simulink model "afe_inv_ttype_psm"  (R2026a)
settings: Solver=ode23tb  StopTime=simlength  FixedStep=tc  MaxStep=glb_time.tc
values from neighbouring files (symbols this model uses):
  afe_ctrl = ctrl_afe_setup(glb_time.ts_afe, grid_emu.omega_grid_nom)    [init_model.m]
  afe_pwm_phase_shift_mod1 = 0    [init_model.m]
  DThs_init = 0    [init_model.m]
  filters = setup_global_filters(glb_time.ts_afe, glb_time.ts_inv, glb_time.ts_dab, glb_time.tc)    [init_model.m]
  frt_data = frt_settings(test_index, test_subindex, asymmetric_error_type,      enable_frt_1, enable_frt_2, start_time_LVRT, deepPOSxi, deepPOSeta, deepNEGxi, deepNEGeta)    [init_model.m]
  glb_time = timing_setup(fpwm_afe, trgo_afe, fpwm_inv, trgo_inv, fpwm_single_phase_inv, trgo_single_phase_inv, fpwm_dab, trgo_dab,      fpwm_psfbc, trgo_psfbc, fpwm_isop_rail, trgo_isop_rail, fpwm_cllc, trgo_cllc, t_measure, tc_factor, tc_decimation, delay_pwm, dead_time_afe,      dead_time_inv, dead_time_single_phase_inv, dead_time_dab, dead_time_psfbc, dead_time_isop_rail, dead_time_cllc)    [init_model.m]
  grid_emu = grid_three_phase_emulator('Dyn11', delta_star, grid_nominal_power, application_voltage, us1, us2, fgrid,                  eq_grid_inductance, eq_grid_resistance, eta, ucc, i1m, p_iron, n1, n2, core_area, core_length, mur,                  up_xi_pu_ref, up_eta_pu_ref, un_xi_pu_ref, un_eta_pu_ref)    [init_model.m]
  i_react_pos_ref_2 = -ixi_ref_mod1*tan(acos(0.95))    [init_model.m]
  i_react_pos_ref_3 = ixi_ref_mod1*tan(acos(0.95))    [init_model.m]
  ixi_ref_mod1 = -0.85    [init_model.m]
  ki_align = 18    [init_model.m]
  kp_align = 0.25    [init_model.m]
  lim_down_align = -0.05    [init_model.m]
  lim_up_align = 0.05    [init_model.m]
  mavarage_filter_frequency_base_order = 2    [init_model.m]
  omega_m_sim = psm.omega_m_bez    [init_model.m]
  psm = psm_calculus()    [init_model.m]
  psm_ctrl = ctrl_pmsm_setup(glb_time.ts_inv, psm.omega_bez, u_psm_scale, psm.Jm_norm)    [init_model.m]
  simlength = 1.75    [init_model.m]
  Tambient = 40    [init_model.m]
  time_aux_power_supply_fault = 1e3    (= 1000)    [init_model.m]
  time_gain_afe_module_1 = 1.0002    [init_model.m]
  time_gain_inv_module_2 = 1.001    [init_model.m]
  time_i_react_pos_ref_1 = start_time_LVRT + error_length + 0.335    [init_model.m]
  time_i_react_pos_ref_2 = time_i_react_pos_ref_1 + 0.5    (= 0.5)    [init_model.m]
  time_start_motor_control = 0.25    [init_model.m]
  torque_overload_factor = 1    [init_model.m]
  u_cm_comp_mod1 = 0    [init_model.m]
  u_psm_scale_ekf = sqrt(3)/2 * 2/3 * hwdata.inv.udc_nom/psm.ubez    [init_model.m]
undefined symbols (not defined in the file or in its folder): hwdata, magnitude, omega_m_bez, rpm_base, torque_base
libraries: fl_lib x74, nesl_utility x43, moving_average_filter x10, moving_average_filter_cc x8, discrete_time_low_pass_filter x4, sl_discontinuities x3, single_phase_transformer_lib x3, linear_double_integrator_observer_ccaller x2, threephase_inductor_lib x2, dclink_for_three_levels x2, three_phase_three_level_ttype_inverter_ideal_switch_based_model x2, cstblocks_lti x2
(part 6 of 9)

== system afe_inv_ttype_psm/afe_abc_inv_psm_mod1/AFE_control/afe_control/grid_voltage_phase_lock_loops/dq_pll_ccaller/first_harmonic_tracker_phase_u ==
  u : Inport
  Bus Selector : BusSelector  OutputSignals=output_pu_hat
  C Caller : CCaller  FunctionName=first_harmonic_tracker_process_simulink  PortSpecificationStruct="%)30     .    B \\   8    (     @         %    \"     D    !     0         %  0 \"0    $    _    07)G3F%M90  4&]R=$YA;64 4V-O<&4     26YD97@     5'EP90      4VEZ90      27-';&]B86P   X    P    !@    @    $          4    (     0    ,    !         !   P!O=70 #@   #     &    \"     0         !0    @    !     P    $         $  # &]U=  .    .     8    (    !          %    \"     $    &     0         0  ...(+4988 chars)"
  Constant : Constant  Value=glb_time.ts_afe
  Constant1 : Constant  Value=0
  Constant4 : Constant  Value=afe_ctrl.fht_grid.omega_fht
  Constant5 : Constant  Value=afe_ctrl.fht_grid.delta_fht
  Constant6 : Constant  Value=afe_ctrl.fht_grid.Ld_fht(1)
  Constant7 : Constant  Value=afe_ctrl.fht_grid.Ld_fht(2)
  Data Type Conversion{1..2,6..9} (6 alike) : DataTypeConversion  OutDataTypeStr=single  SaturateOnIntegerOverflow=off  RndMeth=Floor
  Data Type Conversion3 : DataTypeConversion  OutDataTypeStr=uint8  SaturateOnIntegerOverflow=off  RndMeth=Floor
  Data Type Conversion4 : DataTypeConversion  OutDataTypeStr=double  SaturateOnIntegerOverflow=off  RndMeth=Floor
  Data Type Conversion5 : DataTypeConversion  OutDataTypeStr=uint8  SaturateOnIntegerOverflow=off  RndMeth=Floor
  Step : Step  Time=0.0125  InitialValue=1  FinalValue=0
  u_hat : Outport
  wires:
  Data Type Conversion4/1 -> u_hat/1
  Data Type Conversion3/1 -> C Caller/1
  Data Type Conversion1/1 -> C Caller/3
  Data Type Conversion2/1 -> C Caller/2
  C Caller/1 -> Bus Selector/1
  Bus Selector/1 -> Data Type Conversion4/1  "<output_pu_hat>"
  Step/1 -> Data Type Conversion3/1
  u/1 -> Data Type Conversion2/1
  Constant/1 -> Data Type Conversion1/1
  Constant1/1 -> Data Type Conversion5/1
  Constant4/1 -> Data Type Conversion6/1
  Constant6/1 -> Data Type Conversion8/1
  Constant7/1 -> Data Type Conversion9/1
  Constant5/1 -> Data Type Conversion7/1
  Data Type Conversion5/1 -> C Caller/8
  Data Type Conversion6/1 -> C Caller/4
  Data Type Conversion7/1 -> C Caller/5
  Data Type Conversion8/1 -> C Caller/6
  Data Type Conversion9/1 -> C Caller/7

== system afe_inv_ttype_psm/afe_abc_inv_psm_mod1/AFE_control/afe_control/grid_voltage_phase_lock_loops/dq_pll_ccaller/first_harmonic_tracker_phase_v ==
  u : Inport
  Bus Selector : BusSelector  OutputSignals=output_pu_hat
  C Caller : CCaller  FunctionName=first_harmonic_tracker_process_simulink  PortSpecificationStruct="%)30     .    B \\   8    (     @         %    \"     D    !     0         %  0 \"0    $    _    07)G3F%M90  4&]R=$YA;64 4V-O<&4     26YD97@     5'EP90      4VEZ90      27-';&]B86P   X    P    !@    @    $          4    (     0    ,    !         !   P!O=70 #@   #     &    \"     0         !0    @    !     P    $         $  # &]U=  .    .     8    (    !          %    \"     $    &     0         0  ...(+4988 chars)"
  Constant : Constant  Value=glb_time.ts_afe
  Constant1 : Constant  Value=2
  Constant4 : Constant  Value=afe_ctrl.fht_grid.omega_fht
  Constant5 : Constant  Value=afe_ctrl.fht_grid.delta_fht
  Constant6 : Constant  Value=afe_ctrl.fht_grid.Ld_fht(1)
  Constant7 : Constant  Value=afe_ctrl.fht_grid.Ld_fht(2)
  Data Type Conversion{1..2,6..9} (6 alike) : DataTypeConversion  OutDataTypeStr=single  SaturateOnIntegerOverflow=off  RndMeth=Floor
  Data Type Conversion3 : DataTypeConversion  OutDataTypeStr=uint8  SaturateOnIntegerOverflow=off  RndMeth=Floor
  Data Type Conversion4 : DataTypeConversion  OutDataTypeStr=double  SaturateOnIntegerOverflow=off  RndMeth=Floor
  Data Type Conversion5 : DataTypeConversion  OutDataTypeStr=uint8  SaturateOnIntegerOverflow=off  RndMeth=Floor
  Step : Step  Time=0.0125  InitialValue=1  FinalValue=0
  u_hat : Outport
  wires:
  Data Type Conversion9/1 -> C Caller/7
  Data Type Conversion8/1 -> C Caller/6
  Data Type Conversion7/1 -> C Caller/5
  Data Type Conversion6/1 -> C Caller/4
  Data Type Conversion5/1 -> C Caller/8
  Constant5/1 -> Data Type Conversion7/1
  Constant7/1 -> Data Type Conversion9/1
  Constant6/1 -> Data Type Conversion8/1
  Constant4/1 -> Data Type Conversion6/1
  Constant1/1 -> Data Type Conversion5/1
  Constant/1 -> Data Type Conversion1/1
  u/1 -> Data Type Conversion2/1
  Step/1 -> Data Type Conversion3/1
  Bus Selector/1 -> Data Type Conversion4/1  "<output_pu_hat>"
  C Caller/1 -> Bus Selector/1
  Data Type Conversion2/1 -> C Caller/2
  Data Type Conversion1/1 -> C Caller/3
  Data Type Conversion3/1 -> C Caller/1
  Data Type Conversion4/1 -> u_hat/1

== system afe_inv_ttype_psm/afe_abc_inv_psm_mod1/AFE_control/afe_control/grid_voltage_phase_lock_loops/dq_pll_ccaller/first_harmonic_tracker_phase_w ==
  u : Inport
  Bus Selector : BusSelector  OutputSignals=output_pu_hat
  C Caller : CCaller  FunctionName=first_harmonic_tracker_process_simulink  PortSpecificationStruct="%)30     .    B \\   8    (     @         %    \"     D    !     0         %  0 \"0    $    _    07)G3F%M90  4&]R=$YA;64 4V-O<&4     26YD97@     5'EP90      4VEZ90      27-';&]B86P   X    P    !@    @    $          4    (     0    ,    !         !   P!O=70 #@   #     &    \"     0         !0    @    !     P    $         $  # &]U=  .    .     8    (    !          %    \"     $    &     0         0  ...(+4988 chars)"
  Constant : Constant  Value=glb_time.ts_afe
  Constant1 : Constant  Value=4
  Constant4 : Constant  Value=afe_ctrl.fht_grid.omega_fht
  Constant5 : Constant  Value=afe_ctrl.fht_grid.delta_fht
  Constant6 : Constant  Value=afe_ctrl.fht_grid.Ld_fht(1)
  Constant7 : Constant  Value=afe_ctrl.fht_grid.Ld_fht(2)
  Data Type Conversion{1..2,6..9} (6 alike) : DataTypeConversion  OutDataTypeStr=single  SaturateOnIntegerOverflow=off  RndMeth=Floor
  Data Type Conversion3 : DataTypeConversion  OutDataTypeStr=uint8  SaturateOnIntegerOverflow=off  RndMeth=Floor
  Data Type Conversion4 : DataTypeConversion  OutDataTypeStr=double  SaturateOnIntegerOverflow=off  RndMeth=Floor
  Data Type Conversion5 : DataTypeConversion  OutDataTypeStr=uint8  SaturateOnIntegerOverflow=off  RndMeth=Floor
  Step : Step  Time=0.0125  InitialValue=1  FinalValue=0
  u_hat : Outport
  wires:
  Data Type Conversion4/1 -> u_hat/1
  Data Type Conversion3/1 -> C Caller/1
  Data Type Conversion1/1 -> C Caller/3
  Data Type Conversion2/1 -> C Caller/2
  C Caller/1 -> Bus Selector/1
  Bus Selector/1 -> Data Type Conversion4/1  "<output_pu_hat>"
  Step/1 -> Data Type Conversion3/1
  u/1 -> Data Type Conversion2/1
  Constant/1 -> Data Type Conversion1/1
  Constant1/1 -> Data Type Conversion5/1
  Constant4/1 -> Data Type Conversion6/1
  Constant6/1 -> Data Type Conversion8/1
  Constant7/1 -> Data Type Conversion9/1
  Constant5/1 -> Data Type Conversion7/1
  Data Type Conversion5/1 -> C Caller/8
  Data Type Conversion6/1 -> C Caller/4
  Data Type Conversion7/1 -> C Caller/5
  Data Type Conversion8/1 -> C Caller/6
  Data Type Conversion9/1 -> C Caller/7

== system afe_inv_ttype_psm/afe_abc_inv_psm_mod1/AFE_control/afe_control/grid_voltage_sequences/voltage_sequence_avg/average_filter ==
  v_grid_pos_xi : Inport
  v_grid_pos_eta : Inport  Port=2
  v_grid_neg_xi : Inport  Port=3
  v_grid_neg_eta : Inport  Port=4
  Abs : Abs  SaturateOnIntegerOverflow=off
  Gain : Gain  Gain=grid_emu.omega_grid_nom*mavarage_filter_frequency_base_order
  Saturation : Saturate  UpperLimit=2  LowerLimit=0.1
  dmavg_flt{,1..3} (4 alike) : moving_average_filter/dmavg_flt  ts=glb_time.ts_afe  enable_time=dmavg_filter_enable_time
  v_grid_pos_xi_avg : Outport
  v_grid_pos_eta_avg : Outport  Port=2
  v_grid_neg_xi_avg : Outport  Port=3
  v_grid_neg_eta_avg : Outport  Port=4
  wires:
  v_grid_neg_eta/1 -> dmavg_flt3/1
  v_grid_neg_xi/1 -> dmavg_flt2/1
  v_grid_pos_eta/1 -> dmavg_flt1/1
  dmavg_flt3/1 -> v_grid_neg_eta_avg/1
  dmavg_flt2/1 -> v_grid_neg_xi_avg/1
  dmavg_flt1/1 -> v_grid_pos_eta_avg/1
  Gain/1 -> dmavg_flt/2, dmavg_flt1/2, dmavg_flt2/2, dmavg_flt3/2
  dmavg_flt/1 -> v_grid_pos_xi_avg/1
  v_grid_pos_xi/1 -> dmavg_flt/1
  Abs/1 -> Saturation/1
  [omega_grid_pll_pu] -> Abs/1
  Saturation/1 -> Gain/1

== system afe_inv_ttype_psm/afe_abc_inv_psm_mod1/AFE_control/afe_control/grid_voltage_sequences/voltage_sequence_avg/average_filter_ccaller ==
  v_grid_pos_xi : Inport
  v_grid_pos_eta : Inport  Port=2
  v_grid_neg_xi : Inport  Port=3
  v_grid_neg_eta : Inport  Port=4
  Abs : Abs  SaturateOnIntegerOverflow=off
  Gain : Gain  Gain=grid_emu.omega_grid_nom*mavarage_filter_frequency_base_order
  Saturation : Saturate  UpperLimit=2  LowerLimit=0.1
  dmavg_flt : moving_average_filter_cc/dmavg_flt  instance=0  ts=glb_time.ts_afe  enable_time=dmavg_filter_enable_time
  dmavg_flt1 : moving_average_filter_cc/dmavg_flt  instance=1  ts=glb_time.ts_afe  enable_time=dmavg_filter_enable_time
  dmavg_flt2 : moving_average_filter_cc/dmavg_flt  instance=2  ts=glb_time.ts_afe  enable_time=dmavg_filter_enable_time
  dmavg_flt3 : moving_average_filter_cc/dmavg_flt  instance=3  ts=glb_time.ts_afe  enable_time=dmavg_filter_enable_time
  v_grid_pos_xi_avg : Outport
  v_grid_pos_eta_avg : Outport  Port=2
  v_grid_neg_xi_avg : Outport  Port=3
  v_grid_neg_eta_avg : Outport  Port=4
  wires:
  v_grid_pos_xi/1 -> dmavg_flt/1
  dmavg_flt/1 -> v_grid_pos_xi_avg/1
  dmavg_flt1/1 -> v_grid_pos_eta_avg/1
  dmavg_flt2/1 -> v_grid_neg_xi_avg/1
  dmavg_flt3/1 -> v_grid_neg_eta_avg/1
  v_grid_pos_eta/1 -> dmavg_flt1/1
  v_grid_neg_xi/1 -> dmavg_flt2/1
  v_grid_neg_eta/1 -> dmavg_flt3/1
  Abs/1 -> Saturation/1
  Saturation/1 -> Gain/1
  [omega_grid_pll_pu] -> Abs/1
  Gain/1 -> dmavg_flt/2, dmavg_flt1/2, dmavg_flt3/2, dmavg_flt2/2

== system afe_inv_ttype_psm/afe_abc_inv_psm_mod1/AFE_control/afe_control/phase_compensation_1/alignment_eval_afe1/pi ==
  u_ref : Inport
  u : Inport  Port=2
  1/Ti : Gain  Gain=kp  SaturateOnIntegerOverflow=on  OutDataTypeStr=Inherit: Same as input  ParamDataTypeStr=Inherit: Same as input
  Saturation : Saturate  UpperLimit=lim_up  LowerLimit=lim_down
  Sum1 : Sum  Inputs=+++  SaturateOnIntegerOverflow=on
  Sum2 : Sum  Inputs=-+  SaturateOnIntegerOverflow=on
  Sum3 : Sum  Inputs=-+  SaturateOnIntegerOverflow=on
  Unit Delay4 : UnitDelay  SampleTime=-1
  kp : Gain  Gain=ki  SaturateOnIntegerOverflow=on  OutDataTypeStr=Inherit: Same as input  ParamDataTypeStr=Inherit: Same as input
  y : Outport
  wires:
  1/Ti/1 -> Sum1/1, Sum3/1
  kp/1 -> Sum1/2
  Sum3/1 -> Unit Delay4/1
  Unit Delay4/1 -> Sum1/3
  u_ref/1 -> Sum2/2
  u/1 -> Sum2/1
  Sum2/1 -> kp/1, 1/Ti/1
  Sum1/1 -> Saturation/1
  Saturation/1 -> Sum3/2, y/1

== system afe_inv_ttype_psm/afe_abc_inv_psm_mod1/inv_psm_mod1/inverter/deadtime_generator_for_ttype/dead_time_generator_cmos_simulink_phu/dead_time_leg_generator_1 ==
  cmd_in_QA : Inport
  cmd_in_QB : Inport  Port=2
  MATLAB Function : MATLAB Function  TreatAsAtomicUnit=on
  MATLAB Function1 : MATLAB Function  TreatAsAtomicUnit=on
  MATLAB Function2 : MATLAB Function  TreatAsAtomicUnit=on
  MATLAB Function3 : MATLAB Function  TreatAsAtomicUnit=on
  MATLAB Function4 : MATLAB Function  TreatAsAtomicUnit=on
  MATLAB Function5 : MATLAB Function  TreatAsAtomicUnit=on
  MATLAB Function6 : MATLAB Function  TreatAsAtomicUnit=on
  MATLAB Function7 : MATLAB Function  TreatAsAtomicUnit=on
  MATLAB Function8 : MATLAB Function  TreatAsAtomicUnit=on
  MATLAB Function9 : MATLAB Function  TreatAsAtomicUnit=on
  Transfer Fcn : TransferFcn  Denominator=[sqrt(2)*deadtime 1]
  Transfer Fcn1 : TransferFcn  Denominator=[sqrt(2)*deadtime 1]
  cmd_out_QA : Outport
  cmd_out_QB : Outport  Port=2
  wires:
  MATLAB Function8/1(y) -> MATLAB Function5/2(u2)
  MATLAB Function7/1(y) -> Transfer Fcn1/1, MATLAB Function9/2(u2)
  MATLAB Function3/1(y) -> MATLAB Function1/2(u2)
  MATLAB Function2/1(y) -> Transfer Fcn/1, MATLAB Function4/1(u1)
  MATLAB Function/1(y) -> MATLAB Function1/1(u1), MATLAB Function2/1(u)
  MATLAB Function9/1(y) -> cmd_out_QB/1
  MATLAB Function4/1(y) -> cmd_out_QA/1
  MATLAB Function6/1(y) -> MATLAB Function5/1(u1), MATLAB Function7/1(u)
  cmd_in_QA/1 -> MATLAB Function/1(u)
  MATLAB Function5/1(y) -> MATLAB Function4/2(u2)
  MATLAB Function1/1(y) -> MATLAB Function9/1(u1)
  cmd_in_QB/1 -> MATLAB Function6/1(u)
  Transfer Fcn1/1 -> MATLAB Function8/1(u)
  Transfer Fcn/1 -> MATLAB Function3/1(u)

== system afe_inv_ttype_psm/afe_abc_inv_psm_mod1/inv_psm_mod1/inverter/deadtime_generator_for_ttype/dead_time_generator_cmos_simulink_phv/dead_time_leg_generator_1 ==
  cmd_in_QA : Inport
  cmd_in_QB : Inport  Port=2
  MATLAB Function : MATLAB Function  TreatAsAtomicUnit=on
  MATLAB Function1 : MATLAB Function  TreatAsAtomicUnit=on
  MATLAB Function2 : MATLAB Function  TreatAsAtomicUnit=on
  MATLAB Function3 : MATLAB Function  TreatAsAtomicUnit=on
  MATLAB Function4 : MATLAB Function  TreatAsAtomicUnit=on
  MATLAB Function5 : MATLAB Function  TreatAsAtomicUnit=on
  MATLAB Function6 : MATLAB Function  TreatAsAtomicUnit=on
  MATLAB Function7 : MATLAB Function  TreatAsAtomicUnit=on
  MATLAB Function8 : MATLAB Function  TreatAsAtomicUnit=on
  MATLAB Function9 : MATLAB Function  TreatAsAtomicUnit=on
  Transfer Fcn : TransferFcn  Denominator=[sqrt(2)*deadtime 1]
  Transfer Fcn1 : TransferFcn  Denominator=[sqrt(2)*deadtime 1]
  cmd_out_QA : Outport
  cmd_out_QB : Outport  Port=2
  wires:
  Transfer Fcn/1 -> MATLAB Function3/1(u)
  Transfer Fcn1/1 -> MATLAB Function8/1(u)
  cmd_in_QB/1 -> MATLAB Function6/1(u)
  MATLAB Function1/1(y) -> MATLAB Function9/1(u1)
  MATLAB Function5/1(y) -> MATLAB Function4/2(u2)
  cmd_in_QA/1 -> MATLAB Function/1(u)
  MATLAB Function6/1(y) -> MATLAB Function7/1(u), MATLAB Function5/1(u1)
  MATLAB Function4/1(y) -> cmd_out_QA/1
  MATLAB Function9/1(y) -> cmd_out_QB/1
  MATLAB Function/1(y) -> MATLAB Function2/1(u), MATLAB Function1/1(u1)
  MATLAB Function2/1(y) -> MATLAB Function4/1(u1), Transfer Fcn/1
  MATLAB Function3/1(y) -> MATLAB Function1/2(u2)
  MATLAB Function7/1(y) -> MATLAB Function9/2(u2), Transfer Fcn1/1
  MATLAB Function8/1(y) -> MATLAB Function5/2(u2)

== system afe_inv_ttype_psm/afe_abc_inv_psm_mod1/inv_psm_mod1/inverter/deadtime_generator_for_ttype/dead_time_generator_cmos_simulink_phw/dead_time_leg_generator_1 ==
  cmd_in_QA : Inport
  cmd_in_QB : Inport  Port=2
  MATLAB Function : MATLAB Function  TreatAsAtomicUnit=on
  MATLAB Function1 : MATLAB Function  TreatAsAtomicUnit=on
  MATLAB Function2 : MATLAB Function  TreatAsAtomicUnit=on
  MATLAB Function3 : MATLAB Function  TreatAsAtomicUnit=on
  MATLAB Function4 : MATLAB Function  TreatAsAtomicUnit=on
  MATLAB Function5 : MATLAB Function  TreatAsAtomicUnit=on
  MATLAB Function6 : MATLAB Function  TreatAsAtomicUnit=on
  MATLAB Function7 : MATLAB Function  TreatAsAtomicUnit=on
  MATLAB Function8 : MATLAB Function  TreatAsAtomicUnit=on
  MATLAB Function9 : MATLAB Function  TreatAsAtomicUnit=on
  Transfer Fcn : TransferFcn  Denominator=[sqrt(2)*deadtime 1]
  Transfer Fcn1 : TransferFcn  Denominator=[sqrt(2)*deadtime 1]
  cmd_out_QA : Outport
  cmd_out_QB : Outport  Port=2
  wires:
  MATLAB Function8/1(y) -> MATLAB Function5/2(u2)
  MATLAB Function7/1(y) -> Transfer Fcn1/1, MATLAB Function9/2(u2)
  MATLAB Function3/1(y) -> MATLAB Function1/2(u2)
  MATLAB Function2/1(y) -> Transfer Fcn/1, MATLAB Function4/1(u1)
  MATLAB Function/1(y) -> MATLAB Function1/1(u1), MATLAB Function2/1(u)
  MATLAB Function9/1(y) -> cmd_out_QB/1
  MATLAB Function4/1(y) -> cmd_out_QA/1
  MATLAB Function6/1(y) -> MATLAB Function5/1(u1), MATLAB Function7/1(u)
  cmd_in_QA/1 -> MATLAB Function/1(u)
  MATLAB Function5/1(y) -> MATLAB Function4/2(u2)
  MATLAB Function1/1(y) -> MATLAB Function9/1(u1)
  cmd_in_QB/1 -> MATLAB Function6/1(u)
  Transfer Fcn1/1 -> MATLAB Function8/1(u)
  Transfer Fcn/1 -> MATLAB Function3/1(u)

== system afe_inv_ttype_psm/afe_abc_inv_psm_mod1/inv_psm_mod1/inverter_ctrl/inverter_control/encoder-sensorless-switch/double_integrator_observer ==
  phase_psm : Inport
  Dead Zone : DeadZone  LowerValue=-0.01  UpperValue=0.01
  Gain : Gain  Gain=psm_ctrl.di_obs.komega
  Gain1 : Gain  Gain=psm_ctrl.di_obs.ktheta
  Gain2 : Gain  Gain=psm_ctrl.omega_base
  Gain3 : Gain  Gain=1/psm_ctrl.omega_base
  Gain4 : Gain  Gain=glb_time.ts_inv
  Gain5 : Gain  Gain=glb_time.ts_inv
  Gain6 : Gain  Gain=glb_time.ts_inv
  Sum : Sum  Inputs=-+|
  Sum1 : Sum  Inputs=|++
  Sum2 : Sum  Inputs=|++
  Sum8 : Sum  Inputs=++|
  Unit Delay1 : UnitDelay  InitialCondition=pi  SampleTime=-1
  Unit Delay2 : UnitDelay  SampleTime=-1
  bounder1 : MATLAB Function  TreatAsAtomicUnit=on
  bounder2 : MATLAB Function  TreatAsAtomicUnit=on
  omega_pu_psm_hat : Outport  VectorParamsAs1DForOutWhenUnconnected=off
  phase_psm_hat : Outport  Port=2  VectorParamsAs1DForOutWhenUnconnected=off
  wires:
  Gain1/1 -> Gain6/1
  phase_psm/1 -> Sum/2
  Sum8/1 -> Unit Delay1/1
  Unit Delay1/1 -> bounder2/1(u)
  Sum1/1 -> Unit Delay2/1
  Gain/1 -> Gain4/1
  Unit Delay2/1 -> omega_pu_psm_hat/1, Sum1/2, Gain5/1
  Sum2/1 -> Sum8/2
  bounder2/1(y) -> Sum2/2, phase_psm_hat/1, Sum/1  "phase_hat"
  bounder1/1(y) -> Gain1/1, Gain/1
  Gain2/1 -> Sum8/1
  Gain3/1 -> Sum1/1
  Gain5/1 -> Gain2/1
  Sum/1 -> bounder1/1(u)
  Gain4/1 -> Gain3/1
  Gain6/1 -> Sum2/1

== system afe_inv_ttype_psm/afe_abc_inv_psm_mod1/inv_psm_mod1/inverter_ctrl/inverter_control/inner_ctrl/bemf_observer1 ==
  ialpha_pu : Inport
  ibeta_pu : Inport  Port=2
  ualpha_pu : Inport  Port=3
  ubeta_pu : Inport  Port=4
  udc_pu : Inport  Port=5
  EKF_bemf_observer : Subsystem
  Mux : Mux
  Mux1 : Mux
  Observer Comparison mod1 : Scope  NumInputPorts=2
      settings: ActiveDisplayYMinimum=-1.7949249844307968  ActiveDisplayYMaximum=1.3113178143582995
  Variant Source1 : VariantSource  VariantControls={use_ekf_bemf_module_1 == 1, use_observer_from_simulink_module_1 == 1, use_observer_from_ccaller_module_1 == 1}
  Variant Source2 : VariantSource  VariantControls={use_ekf_bemf_module_1 == 1, use_observer_from_simulink_module_1 == 1, use_observer_from_ccaller_module_1 == 1}
  bemf_observer : Subsystem
  bemf_observer_ccaller : Subsystem
  tag scope: omega_hat_pu_mod1=scoped, phase_hat_mod1=scoped
  wires:
  ialpha_pu/1 -> EKF_bemf_observer/1(ialpha_pu), bemf_observer_ccaller/1(ialpha_pu), bemf_observer/1(ialpha_pu)
  ibeta_pu/1 -> EKF_bemf_observer/2(ibeta_pu), bemf_observer_ccaller/2(ibeta_pu), bemf_observer/2(ibeta_pu)
  Mux/1 -> Observer Comparison mod1/1
  Mux1/1 -> Observer Comparison mod1/2
  ualpha_pu/1 -> EKF_bemf_observer/3(ualpha_pu), bemf_observer_ccaller/3(ualpha_pu), bemf_observer/3(ualpha_pu)
  ubeta_pu/1 -> EKF_bemf_observer/4(ubeta_pu), bemf_observer_ccaller/4(ubeta_pu), bemf_observer/4(ubeta_pu)
  Variant Source1/1 -> [phase_hat_mod1]
  Variant Source2/1 -> [omega_hat_pu_mod1]
  udc_pu/1 -> EKF_bemf_observer/5(udc_pu), bemf_observer_ccaller/5(udc_pu), bemf_observer/5(udc_pu)
  [omegad_pu_psm] -> Mux/4  "omega_pu_psm"
  [phased_psm] -> Mux1/4  "phase_psm"
  EKF_bemf_observer/2(omega_elec_ekf_hat) -> [omega_elec_ekf_hat]  "omega_elec_ekf_hat"
  EKF_bemf_observer/1(phase_elec_ekf_hat) -> [phase_elec_ekf_hat]  "phase_elec_ekf_hat"
  bemf_observer/1(omega_pu) -> [omega_elec_bemf_hat]  "omega_elec_bemf_hat"
  bemf_observer/2(theta_hat) -> [phase_elec_bemf_hat]  "phase_elec_bemf_hat"
  bemf_observer_ccaller/2(theta_hat) -> [phase_elec_bemf_cc_hat]  "phase_elec_bemf_cc_hat"
  bemf_observer_ccaller/1(omega_pu) -> [omega_elec_bemf_cc_hat]  "omega_elec_bemf_cc_hat"
  [phase_elec_bemf_cc_hat] -> Mux1/3  "phase_bemf_cc_hat"
  [omega_elec_bemf_cc_hat] -> Mux/3  "omega_bemf_cc_hat"
  [omega_elec_bemf_hat] -> Mux/2  "omega_bemf_hat"
  [phase_elec_bemf_hat] -> Mux1/2  "phase_bemf_hat"
  [phase_elec_ekf_hat] -> Mux1/1  "phase_ekf_hat"
  [omega_elec_ekf_hat] -> Mux/1  "omega_ekf_hat"
  [omega_elec_ekf_hat] -> Variant Source2/1
  [omega_elec_bemf_hat] -> Variant Source2/2
  [omega_elec_bemf_cc_hat] -> Variant Source2/3
  [phase_elec_ekf_hat] -> Variant Source1/1
  [phase_elec_bemf_hat] -> Variant Source1/2
  [phase_elec_bemf_cc_hat] -> Variant Source1/3

== system afe_inv_ttype_psm/afe_abc_inv_psm_mod1/inv_psm_mod1/inverter_ctrl/inverter_control/inner_ctrl/current_reference_generator ==
  torque_ref_pu : Inport
  theta_elec_hat : Inport  Port=2
  Gain5 : Gain  Gain=-1
  Product : Product
  Product1 : Product
  Trigonometric Function1 : Trigonometry
  Trigonometric Function2 : Trigonometry  Operator=cos
  i_alpha_ref : Outport
  i_beta_ref : Outport  Port=2
  tag scope: ialpha_pu_ref_mod1=scoped, ibeta_pu_ref_mod1=scoped
  wires:
  Trigonometric Function1/1 -> Product/2
  Product1/1 -> [ibeta_pu_ref_mod1], i_beta_ref/1
  Trigonometric Function2/1 -> Product1/2
  Product/1 -> Gain5/1
  Gain5/1 -> [ialpha_pu_ref_mod1], i_alpha_ref/1
  torque_ref_pu/1 -> Product/1, Product1/1
  theta_elec_hat/1 -> Trigonometric Function1/1, Trigonometric Function2/1  "theta_electrical"

== system afe_inv_ttype_psm/afe_abc_inv_psm_mod1/inv_psm_mod1/inverter_ctrl/inverter_control/inner_ctrl/current_transformation ==
  Demux : Demux  Outputs=3
  alphabeta2dq : MATLAB Function  TreatAsAtomicUnit=on
  uvw2alphabeta : MATLAB Function  TreatAsAtomicUnit=on
  tag scope: ialpha_pu_mod1=global, ibeta_pu_mod1=global, id_pu_mod1=global, iq_pu_mod1=global
  wires:
  alphabeta2dq/2(q) -> [iq_pu_mod1]  "iq_pu"
  alphabeta2dq/1(d) -> [id_pu_mod1]  "id_pu"
  uvw2alphabeta/2(beta) -> alphabeta2dq/2(beta), [ibeta_pu_mod1]  "ibeta_pu"
  uvw2alphabeta/1(alpha) -> [ialpha_pu_mod1], alphabeta2dq/1(alpha)  "ialpha_pu"
  [motor_phase_ctrl_mod1] -> alphabeta2dq/3(gamma)
  Demux/3 -> uvw2alphabeta/3(w)  "iw"
  Demux/2 -> uvw2alphabeta/2(v)  "iv"
  Demux/1 -> uvw2alphabeta/1(u)  "iu"
  [isd_uvw_inv_mod1] -> Demux/1

== system afe_inv_ttype_psm/afe_abc_inv_psm_mod1/inv_psm_mod1/inverter_ctrl/inverter_control/inner_ctrl/mp control ==
  vdc1_pu : Inport
  vdc2_pu : Inport  Port=2
  ialpha_pu_ref : Inport  Port=3
  ialpha_pu : Inport  Port=4
  ibeta_pu_ref : Inport  Port=5
  ibeta_pu : Inport  Port=6
  omega_pu : Inport  Port=7
  psi_alpha_pu_hat : Inport  Port=8
  psi_beta_pu_hat : Inport  Port=9
  Bus Creator : BusCreator  Inputs=4
  Bus Creator1 : BusCreator  Inputs=2
  Bus Creator2 : BusCreator  Inputs=2
  Bus Creator3 : BusCreator  Inputs=3
  Bus Creator4 : BusCreator  Inputs=4
  Bus Creator5 : BusCreator  Inputs=4
  Constant : Constant  Value=psm.Lalpha_norm
  Constant1 : Constant  Value=psm.Rs_norm
  Constant2 : Constant  Value=psm.Lbeta_norm
  Constant3 : Constant  Value=psm.omega_bez
  Constant4 : Constant  Value=psm_ctrl.ekf.k_kalman
  Constant5 : Constant  Value=psm_ctrl.ekf.k_dc
  Constant6 : Constant  Value=psm_ctrl.ekf.k_sw
  Constant7 : Constant  Value=glb_time.ts_inv
  Gain2 : Gain  Gain=3
  Gain3 : Gain  Gain=3
  discrete-time-low-pass-filter : discrete_time_low_pass_filter/discrete-time-low-pass-filter  Commented=through  tau=5e-3  ts=glb_time.ts_inv
  discrete-time-low-pass-filter1 : discrete_time_low_pass_filter/discrete-time-low-pass-filter  Commented=through  tau=5e-3  ts=glb_time.ts_inv
  ialpha/beta_tracking : Scope  NumInputPorts=2
      settings: ActiveDisplayYMinimum=0.087780674058203917  ActiveDisplayYMaximum=0.2221650117076063  DataLoggingVariableName=ScopeData2
  mpc_pu_d : MATLAB Function  TreatAsAtomicUnit=on
  ualpha : Outport
  ubeta : Outport  Port=2
  cmd_gates : Outport  Port=3
  wires:
  ialpha_pu_ref/1 -> Bus Creator1/1, mpc_pu_d/3(ialpha_ref)  "ialpha_pu_ref"
  ibeta_pu_ref/1 -> Bus Creator2/1, mpc_pu_d/4(ibeta_ref)  "ibeta_pu_ref"
  ialpha_pu/1 -> Bus Creator1/2, mpc_pu_d/5(ialpha)  "ialpha_pu"
  ibeta_pu/1 -> Bus Creator2/2, mpc_pu_d/6(ibeta)  "ibeta_pu"
  omega_pu/1 -> mpc_pu_d/7(omega_hat)  "omega_hat"
  psi_alpha_pu_hat/1 -> mpc_pu_d/8(psi_alpha_hat)  "psi_alpha_hat"
  psi_beta_pu_hat/1 -> mpc_pu_d/9(psi_beta_hat)  "psi_beta_hat"
  vdc1_pu/1 -> mpc_pu_d/1(vdc1)
  Bus Creator1/1 -> ialpha/beta_tracking/1
  Bus Creator2/1 -> ialpha/beta_tracking/2
  Bus Creator3/1 -> cmd_gates/1
  Bus Creator4/1 -> Bus Creator3/2  "gate_cmds_phv"
  mpc_pu_d/12(S4c) -> Bus Creator5/4  "cmd_gate_Q4"
  mpc_pu_d/5(S1b) -> Bus Creator4/1  "cmd_gate_Q1"
  mpc_pu_d/9(S1c) -> Bus Creator5/1  "cmd_gate_Q1"
  Bus Creator5/1 -> Bus Creator3/3  "gate_cmds_phw"
  mpc_pu_d/4(S4a) -> Bus Creator/4  "cmd_gate_Q4"
  mpc_pu_d/6(S2b) -> Bus Creator4/2  "cmd_gate_Q2"
  mpc_pu_d/1(S1a) -> Bus Creator/1  "cmd_gate_Q1"
  mpc_pu_d/7(S3b) -> Bus Creator4/3  "cmd_gate_Q3"
  mpc_pu_d/3(S3a) -> Bus Creator/3  "cmd_gate_Q3"
  mpc_pu_d/11(S3c) -> Bus Creator5/3  "cmd_gate_Q3"
  mpc_pu_d/2(S2a) -> Bus Creator/2  "cmd_gate_Q2"
  Bus Creator/1 -> Bus Creator3/1  "gate_cmds_phu"
  mpc_pu_d/10(S2c) -> Bus Creator5/2  "cmd_gate_Q2"
  mpc_pu_d/8(S4b) -> Bus Creator4/4  "cmd_gate_Q4"
  vdc2_pu/1 -> mpc_pu_d/2(vdc2)
  mpc_pu_d/13(ualpha) -> Gain3/1
  mpc_pu_d/14(ubeta) -> Gain2/1
  discrete-time-low-pass-filter/1 -> ualpha/1
  discrete-time-low-pass-filter1/1 -> ubeta/1
  Gain2/1 -> discrete-time-low-pass-filter1/1
  Gain3/1 -> discrete-time-low-pass-filter/1
  Constant/1 -> mpc_pu_d/10(Lalpha_norm)
  Constant1/1 -> mpc_pu_d/11(Rs_norm)
  Constant2/1 -> mpc_pu_d/12(Lbeta_norm)
  Constant3/1 -> mpc_pu_d/13(omega_bez)
  Constant4/1 -> mpc_pu_d/14(k_kalman)
  Constant5/1 -> mpc_pu_d/15(k_dc)
  Constant6/1 -> mpc_pu_d/16(k_sw)
  Constant7/1 -> mpc_pu_d/17(ts_inv)

== system afe_inv_ttype_psm/afe_abc_inv_psm_mod1/inv_psm_mod1/inverter_ctrl/inverter_control/is inv quantizzation and one step delay/is inv quantizzation and one step delay ==
  is_u_pu : Inport
  is_v_pu : Inport  Port=2
  is_w_pu : Inport  Port=3
  Gain3 : Gain  Gain=-1
  Gain4 : Gain  Gain=-1
  Gain5 : Gain  Gain=-1
  Quantizer : Quantizer  QuantizationInterval=adc_quantization
  Quantizer1 : Quantizer  QuantizationInterval=adc_quantization
  Quantizer2 : Quantizer  QuantizationInterval=adc_quantization
  Unit Delay : UnitDelay  SampleTime=-1
  Unit Delay1 : UnitDelay  SampleTime=-1
  Unit Delay2 : UnitDelay  SampleTime=-1
  Zero-Order Hold : ZeroOrderHold  SampleTime=-1
  Zero-Order Hold1 : ZeroOrderHold  SampleTime=-1
  Zero-Order Hold2 : ZeroOrderHold  SampleTime=-1
  isd_u_pu : Outport
  isd_v_pu : Outport  Port=2
  isd_w_pu : Outport  Port=3
  wires:
  Unit Delay/1 -> Gain3/1
  Unit Delay1/1 -> Gain4/1
  Unit Delay2/1 -> Gain5/1
  Quantizer/1 -> Unit Delay/1
  Quantizer1/1 -> Unit Delay1/1
  Quantizer2/1 -> Unit Delay2/1
  is_u_pu/1 -> Zero-Order Hold/1
  is_v_pu/1 -> Zero-Order Hold1/1
  is_w_pu/1 -> Zero-Order Hold2/1
  Gain3/1 -> isd_u_pu/1
  Gain4/1 -> isd_v_pu/1
  Gain5/1 -> isd_w_pu/1
  Zero-Order Hold/1 -> Quantizer/1
  Zero-Order Hold1/1 -> Quantizer1/1
  Zero-Order Hold2/1 -> Quantizer2/1

== system afe_inv_ttype_psm/afe_abc_inv_psm_mod1/inv_psm_mod1/inverter_ctrl/inverter_control/omega_pu/flt ==
  input : Inport
  Gain3 : Gain  Gain=filters.inv.g1_1Hz
  Gain6 : Gain  Gain=filters.inv.g0_1Hz
  Sum : Sum  Inputs=|++
  Unit Delay1 : UnitDelay  SampleTime=-1
  output : Outport  VectorParamsAs1DForOutWhenUnconnected=off
  wires:
  Gain6/1 -> Sum/1
  input/1 -> Gain6/1
  Unit Delay1/1 -> Gain3/1
  Gain3/1 -> Sum/2
  Sum/1 -> Unit Delay1/1, output/1

== system afe_inv_ttype_psm/afe_abc_inv_psm_mod1/inv_psm_mod1/inverter_ctrl/inverter_control/phase_compensation_1/alignment_ctrl ==
  local_time : Inport
  master_time : Inport  Port=2
  Constant : Constant  Value=0
  Gain : Gain  Gain=-1
  Sum : Sum  Inputs=|+-
  pi : Subsystem  mask{kp=0 %kp_align, ki=0 %ki_align, lim_up=lim_up_align, lim_down=lim_down_align}
      mask prompts: ki "ki*ts"
      mask Display:
      | disp('pi()');
      | port_label('input', 1, 'u_ref');
      | port_label('input', 2, 'u');
      | port_label('output', 1, 'y');
  dp : Outport
  wires:
  master_time/1 -> Sum/1
  Sum/1 -> Gain/1
  Constant/1 -> pi/1(u_ref)
  local_time/1 -> Sum/2
  Gain/1 -> pi/2(u)
  pi/1(y) -> dp/1

== system afe_inv_ttype_psm/afe_abc_inv_psm_mod1/inv_psm_mod1/inverter_ctrl/inverter_control/speed_reference_generator/flt ==
  input : Inport
  Gain3 : Gain  Gain=filters.inv.g1_1Hz
  Gain6 : Gain  Gain=filters.inv.g0_1Hz
  Sum : Sum  Inputs=|++
  Unit Delay1 : UnitDelay  SampleTime=-1
  output : Outport  VectorParamsAs1DForOutWhenUnconnected=off
  wires:
  Gain6/1 -> Sum/1
  input/1 -> Gain6/1
  Unit Delay1/1 -> Gain3/1
  Gain3/1 -> Sum/2
  Sum/1 -> Unit Delay1/1, output/1

== system afe_inv_ttype_psm/afe_abc_inv_psm_mod1/AFE_control/afe_control/current_ctrl/inner_current_ctrl/zero_current_ctrl/antiwind_up ==
  d_abc : Inport
  Add : Sum
  Bus Creator : BusCreator  Inputs=3
  Constant : Constant  Value=0
  Demux1 : Demux  Outputs=3
  MATLAB Function1 : MATLAB Function  TreatAsAtomicUnit=on
  MATLAB Function2 : MATLAB Function  TreatAsAtomicUnit=on
  Terminator : Terminator
  Unit Delay1 : UnitDelay  SampleTime=-1
  Unit Delay4 : UnitDelay  SampleTime=-1
  Unit Delay5 : UnitDelay  SampleTime=-1
  afe_ictrl_out/afe_ictrl_ff : Scope  NumInputPorts=3
      settings: ActiveDisplayYMinimum=-1.9658551504914019  ActiveDisplayYMaximum=1.8343082532115993  DataLoggingVariableName=ScopeData4
  anti_wind_up : Subsystem
  ualpha_afe : Outport
  ubeta_afe : Outport  Port=2
  wires:
  MATLAB Function1/1(das) -> MATLAB Function2/1(a), Bus Creator/1  "das"
  d_abc/1 -> Add/1, afe_ictrl_out/afe_ictrl_ff/2
  MATLAB Function1/3(dcs) -> MATLAB Function2/3(c), Bus Creator/3  "dcs"
  [v_grid_ff_abc] -> Unit Delay1/1
  Demux1/2 -> MATLAB Function1/2(db)  "db"
  Demux1/3 -> MATLAB Function1/3(dc)  "dc"
  Bus Creator/1 -> afe_ictrl_out/afe_ictrl_ff/1  "ds_abc"
  Unit Delay1/1 -> afe_ictrl_out/afe_ictrl_ff/3  "u_grid_ff_abc_mod1"
  anti_wind_up/1(scaling) -> MATLAB Function1/4(scaling)
  Demux1/1 -> MATLAB Function1/1(da)  "da"
  Add/1 -> Demux1/1  "d_abc_sum"
  MATLAB Function1/2(dbs) -> MATLAB Function2/2(b), Bus Creator/2  "dbs"
  MATLAB Function2/1(alpha) -> Unit Delay4/1  "u_alpha"
  Unit Delay4/1 -> anti_wind_up/1(alpha), ualpha_afe/1  "ualpha_afe"
  MATLAB Function2/2(beta) -> Unit Delay5/1  "u_beta"
  Unit Delay5/1 -> anti_wind_up/2(beta), ubeta_afe/1  "ubeta_afe"
  MATLAB Function2/3(gamma) -> Terminator/1  "u_gamma"
  Constant/1 -> Add/2

== system afe_inv_ttype_psm/afe_abc_inv_psm_mod1/AFE_control/afe_control/current_ctrl/inner_current_ctrl/zero_current_ctrl/iz ==
  Demux : Demux  Outputs=3
  Gain : Gain  Gain=1/3
  Sum : Sum  Inputs=+++
  iz : Outport
  wires:
  Sum/1 -> Gain/1
  Demux/1 -> Sum/1  "is_a"
  [isd_abc_pu] -> Demux/1
  Demux/3 -> Sum/3  "is_c"
  Demux/2 -> Sum/2  "is_b"
  Gain/1 -> iz/1

== system afe_inv_ttype_psm/afe_abc_inv_psm_mod1/AFE_control/afe_control/current_ctrl/inner_current_ctrl/zero_current_ctrl/zero_sequence_current_ctrl ==
  iz : Inport
  1/Ti : Gain  Gain=afe_ctrl.kp_is_z  SaturateOnIntegerOverflow=on  OutDataTypeStr=Inherit: Same as input  ParamDataTypeStr=Inherit: Same as input
  Constant1 : Constant  Value=0
  Gain : Gain
  Saturation : Saturate  UpperLimit=1  LowerLimit=-1
  Sum1 : Sum  Inputs=+++  SaturateOnIntegerOverflow=on
  Sum2 : Sum  Inputs=-+  SaturateOnIntegerOverflow=on
  Sum3 : Sum  Inputs=-+  SaturateOnIntegerOverflow=on
  Unit Delay4 : UnitDelay  SampleTime=-1
  iz_tracking : Scope  NumInputPorts=3
      settings: ActiveDisplayYMinimum=-1  ActiveDisplayYMaximum=1  DataLoggingVariableName=ScopeData8
  kp : Gain  Gain=afe_ctrl.ki_is_z*glb_time.ts_afe  SaturateOnIntegerOverflow=on  OutDataTypeStr=Inherit: Same as input  ParamDataTypeStr=Inherit: Same as input
  ugamma_afe : Outport
  tag scope: iz_ctrl_out=scoped, iz_pu=scoped, iz_pu_ref=scoped
  wires:
  1/Ti/1 -> Sum1/1, Sum3/1
  kp/1 -> Sum1/2
  Sum3/1 -> Unit Delay4/1
  Unit Delay4/1 -> Sum1/3
  Constant1/1 -> [iz_pu_ref], iz_tracking/1, Sum2/2  "iz_pu_ref"
  iz/1 -> [iz_pu], iz_tracking/2, Sum2/1  "iz_pu"
  Sum2/1 -> kp/1, 1/Ti/1
  Sum1/1 -> Saturation/1
  Saturation/1 -> Gain/1, [iz_ctrl_out], iz_tracking/3, Sum3/2  "iz_ctrl_out"
  Gain/1 -> ugamma_afe/1
